simulink model "ssc_hydromech_power_split_cvt_engine_signal_intf"  (R2025a)
settings: Solver=ode23t  StartTime=0.0  StopTime=70  RelTol=1e-3  AbsTol=1e-3
StartFcn:
  | tic
StopFcn:
  | Elapsed_Sim_Time = toc;
  | disp(['Elapsed Sim Time = ' num2str(Elapsed_Sim_Time)]);
undefined symbols (not defined in the file): DiscIntNeverNeededParam, HMPST, K, Lambda, tau, x0
libraries: fl_lib x30, nesl_utility x16, sm_wheel_loader_lib x9, simulink x7, simulink_extras x6, sdl_lib x3
(part 2 of 4)

== system ssc_hydromech_power_split_cvt_engine_signal_intf/CVT/Other/CVT Ratio Ctrl ==
  Ratio (-) : Inport
  CmdVehSpdDir : Inport  Port=2
  HRBCtrl (-) : Inport  Port=3
  MBCtrl (-) : Inport  Port=4
  Bus Creator : BusCreator  Inputs=12
  Clutch Truth Table : Stateflow chart  TreatAsAtomicUnit=on
  Filter : StateSpace  A=-200  C=200  D=0  InitialCondition=HMPST.Ctrl.Swash.XY_A(1,1)/200
  Range Calculation : Subsystem  mask{XY_I=HMPST.Ctrl.Swash.XY_I}
      mask prompts: XY_I "Range Separation Points"
  Saturation : Saturate  UpperLimit=HMPST.DesignReq.MaxCVTOutputSpeed/HMPST.Eng.wTarget  LowerLimit=0  ZeroCross=off
  Swash Ctrl : Lookup_n-D  NumberOfTableDimensions=1  BreakpointsForDimension1=HMPST.Ctrl.Swash.XY_A(:,2)  BeginIndexSearchUsingPreviousIndexResult=on  Table=HMPST.Ctrl.Swash.XY_A(:,1)  InternalRulePriority=Speed  RndMeth=Simplest
  Transfer Fcn : TransferFcn  Denominator=[0.1 1]
  CVT Ctrl : Outport
  wires:
  Ratio (-)/1 -> [ratio], Transfer Fcn/1
  Clutch Truth Table/1(K1Actv) -> Bus Creator/1  "K1"
  Clutch Truth Table/2(K2Actv) -> Bus Creator/2  "K2"
  Clutch Truth Table/3(K3Actv) -> Bus Creator/3  "K3"
  Clutch Truth Table/4(K4Actv) -> Bus Creator/4  "K4"
  Clutch Truth Table/5(KbActv) -> Bus Creator/5  "Kb"
  Clutch Truth Table/6(KvActv) -> Bus Creator/6  "Kv"
  Clutch Truth Table/7(KrActv) -> Bus Creator/7  "Kr"
  Bus Creator/1 -> CVT Ctrl/1  "Ctrl"
  Range Calculation/1(Range (-)) -> Clutch Truth Table/1(Range)
  Saturation/1 -> Range Calculation/1(Ratio (-)), Swash Ctrl/1
  Transfer Fcn/1 -> Saturation/1
  Filter/1 -> Bus Creator/12  "SwashCtrl"
  Swash Ctrl/1 -> Filter/1  "SwashCtrl"
  HRBCtrl (-)/1 -> Bus Creator/8  "HRBCtrl"
  MBCtrl (-)/1 -> Bus Creator/9  "MBCtrl"
  CmdVehSpdDir/1 -> Bus Creator/11, Clutch Truth Table/2(CmdVehSpdDir)  "CmdVehSpdDir"
  [ratio] -> Bus Creator/10  "ratio"

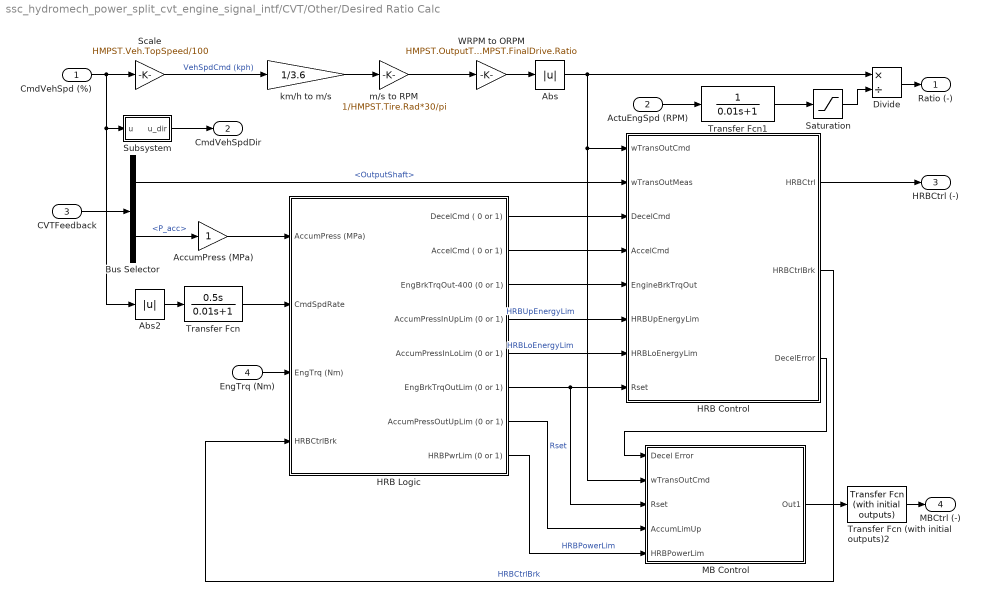
== system ssc_hydromech_power_split_cvt_engine_signal_intf/CVT/Other/Desired Ratio Calc ==
  CmdVehSpd (%) : Inport  SampleTime=HMPST.Simu.TimeStep
  ActuEngSpd (RPM) : Inport  Port=2
  CVTFeedback : Inport  Port=3
  EngTrq (Nm) : Inport  Port=4
  Abs : Abs  ZeroCross=off  SaturateOnIntegerOverflow=off
  Abs2 : Abs  ZeroCross=off  SaturateOnIntegerOverflow=off
  AccumPress (MPa) : Gain
  Bus Selector : BusSelector  OutputSignals=OutputShaft,P_acc
  Divide : Product  Inputs=*/
  HRB Control : Subsystem
  HRB Logic : Subsystem
  MB Control : Subsystem
  Saturation : Saturate  UpperLimit=2500  LowerLimit=0.5
  Scale : Gain  Gain=HMPST.Veh.TopSpeed/100
  Subsystem : Subsystem
  Transfer Fcn : TransferFcn  Numerator=[0.5 0]  Denominator=[0.01 1]
  Transfer Fcn (with initial outputs)2 : simulink_extras/Additional Linear/Transfer Fcn (with initial outputs)  N=1  D=[0.05 1]  Y0=1  U0=1
  Transfer Fcn1 : TransferFcn  Denominator=[0.01 1]
  WRPM to ORPM : Gain  Gain=HMPST.OutputTransferGearPair.Ratio*HMPST.Differential.Ratio*HMPST.FinalDrive.Ratio
  km/h to m/s : Gain  Gain=1/3.6
  m/s to RPM : Gain  Gain=1/HMPST.Tire.Rad*30/pi
  Ratio (-) : Outport
  CmdVehSpdDir : Outport  Port=2
  HRBCtrl (-) : Outport  Port=3
  MBCtrl (-) : Outport  Port=4
  wires:
  MB Control/1(Out1) -> Transfer Fcn (with initial outputs)2/1
  HRB Logic/8(HRBPwrLim (0 or 1)) -> MB Control/5(HRBPowerLim)  "HRBPowerLim"
  HRB Logic/7(AccumPressOutUpLim (0 or 1)) -> MB Control/4(AccumLimUp)
  HRB Control/3(DecelError) -> MB Control/1(Decel Error)
  HRB Control/1(HRBCtrl) -> HRBCtrl (-)/1
  HRB Logic/3(EngBrkTrqOut-400 (0 or 1)) -> HRB Control/5(EngineBrkTrqOut)
  HRB Logic/2(AccelCmd ( 0 or 1)) -> HRB Control/4(AccelCmd)
  HRB Logic/5(AccumPressInLoLim (0 or 1)) -> HRB Control/7(HRBLoEnergyLim)  "HRBLoEnergyLim"
  HRB Logic/4(AccumPressInUpLim (0 or 1)) -> HRB Control/6(HRBUpEnergyLim)  "HRBUpEnergyLim"
  HRB Logic/1(DecelCmd ( 0 or 1)) -> HRB Control/3(DecelCmd)
  Divide/1 -> Ratio (-)/1
  ActuEngSpd (RPM)/1 -> Transfer Fcn1/1
  m/s to RPM/1 -> WRPM to ORPM/1
  km/h to m/s/1 -> m/s to RPM/1
  WRPM to ORPM/1 -> Abs/1
  CmdVehSpd (%)/1 -> Abs2/1, Subsystem/1(u), Scale/1
  Saturation/1 -> Divide/2
  Transfer Fcn1/1 -> Saturation/1
  Bus Selector/1 -> HRB Control/2(wTransOutMeas)  "<OutputShaft>"
  Transfer Fcn/1 -> HRB Logic/2(CmdSpdRate)
  CVTFeedback/1 -> Bus Selector/1
  HRB Logic/6(EngBrkTrqOutLim (0 or 1)) -> MB Control/3(Rset), HRB Control/8(Rset)  "Rset"
  Bus Selector/2 -> AccumPress (MPa)/1  "<P_acc>"
  EngTrq (Nm)/1 -> HRB Logic/3(EngTrq (Nm))
  AccumPress (MPa)/1 -> HRB Logic/1(AccumPress (MPa))
  Subsystem/1(u_dir) -> CmdVehSpdDir/1
  Scale/1 -> km/h to m/s/1  "VehSpdCmd (kph)"
  Abs2/1 -> Transfer Fcn/1
  Abs/1 -> Divide/1, MB Control/2(wTransOutCmd), HRB Control/1(wTransOutCmd)
  Transfer Fcn (with initial outputs)2/1 -> MBCtrl (-)/1
  HRB Control/2(HRBCtrlBrk) -> HRB Logic/4(HRBCtrlBrk)  "HRBCtrlBrk"

== system ssc_hydromech_power_split_cvt_engine_signal_intf/CVT/Other/Port 1 Interface Engine ==
  speed : Inport
  Ideal Rotational Motion Sensor1 : fl_lib/Mechanical/Mechanical Sensors/Ideal Rotational Motion Sensor  reference=foundation.enum.MeasurementReference.difference  acceleration_port=false  velocity_port=true  position_port=true  wrap_angle=simscape.enum.onoff.off  offset=0 rad
  Interface : Subsystem  Variant=on  VariantControlMode=label  VariantControl=Variant1  LabelModeActiveChoice=Continuous
      settings: PortSchema="{\"entries\":[{\"content\":{\"sides\":[{\"content\":{\"connectorIds\":[\"In1\",\"Out2\"]},\"type\":\"ConnectorPlacement.EquallySpacedRectSide\",\"uuid\":\"aa56821c-7799-44e3-b228-553c5b43a68d\"},{\"content\":{\"connectorIds\":[\"In2\",\"Out1\"],\"side\":\"RIGHT\"},\"type\":\"ConnectorPlacement.EquallySpacedRectSide\",\"uuid\":\"8658dee5-55e2-4f33-bdec-e6600ce27fc1\"},{\"content\":{\"connectorIds\":[],\"side\":\"TOP\"},\"type\":\"ConnectorPlacement.EquallySpacedRectSide\",\"uuid\":\"2effe9c6-8e61-4f0c-a39b-329d9ffc707d\"}]},\"type\":\"ConnectorPlacement.EquallySpacedConnector\",\"uuid\":\"c8fc8444-dfc7-49a5-9550-b957635f7d8f\"}],\"packageUris\":[\"http://schema.mathworks.com/mf0/Connector/R2020b\"],\"version\":\"1.0\"}"
  Mechanical Rotational Reference2 : fl_lib/Mechanical/Rotational Elements/Mechanical Rotational Reference
  Mechanical Rotational Reference3 : fl_lib/Mechanical/Rotational Elements/Mechanical Rotational Reference
  T1 : nesl_utility/Simulink-PS Converter  PhysicalDomain=network_engine_domain  SubClassName=ps_input  LeftPortType=input  RightPortType=output  PseudoPeriodic=off  Frequencies=[]  NoiseDistribution=none  NoiseParameters=[]  Unit=N*m  AffineConversion=off  FilteringAndDerivatives=zero  SimscapeFilterOrder=1  InputFilterTimeConstant=0.001  UdotUserProvided=1
  Tau1 : fl_lib/Mechanical/Mechanical Sources/Ideal Torque Source
  w1 : nesl_utility/PS-Simulink Converter  PhysicalDomain=network_engine_domain  SubClassName=ps_output  LeftPortType=input  RightPortType=output  PseudoPeriodic=off  Frequencies=[]  VectorFormat=1-D array  Unit=rad/s  AffineConversion=off
  1 : PMIOPort  Side=Left
  torque : Outport
  wires:
  speed/1 -> Interface/2(across2)
  Interface/2(through1) -> T1/1
  w1/1 -> Interface/1(across1)
  Interface/1(through2) -> torque/1
  connections:
  1/RConn1 -- Ideal Rotational Motion Sensor1/LConn1 -- Tau1/RConn2
  Mechanical Rotational Reference2/LConn1 -- Ideal Rotational Motion Sensor1/RConn1
  Ideal Rotational Motion Sensor1/RConn2 -- w1/LConn1
  Mechanical Rotational Reference3/LConn1 -- Tau1/LConn1
  T1/RConn1 -- Tau1/RConn1

== system ssc_hydromech_power_split_cvt_engine_signal_intf/CVT/Other/Port 1 Interface Vehicle ==
  speed : Inport
  Ideal Rotational Motion Sensor1 : fl_lib/Mechanical/Mechanical Sensors/Ideal Rotational Motion Sensor  reference=foundation.enum.MeasurementReference.difference  acceleration_port=false  velocity_port=true  position_port=true  wrap_angle=simscape.enum.onoff.off  offset=0 rad
  Interface : Subsystem  Variant=on  VariantControlMode=label  VariantControl=Variant1  LabelModeActiveChoice=Continuous
      settings: PortSchema="{\"entries\":[{\"content\":{\"sides\":[{\"content\":{\"connectorIds\":[\"In1\",\"Out2\"]},\"type\":\"ConnectorPlacement.EquallySpacedRectSide\",\"uuid\":\"aa56821c-7799-44e3-b228-553c5b43a68d\"},{\"content\":{\"connectorIds\":[\"In2\",\"Out1\"],\"side\":\"RIGHT\"},\"type\":\"ConnectorPlacement.EquallySpacedRectSide\",\"uuid\":\"8658dee5-55e2-4f33-bdec-e6600ce27fc1\"},{\"content\":{\"connectorIds\":[],\"side\":\"TOP\"},\"type\":\"ConnectorPlacement.EquallySpacedRectSide\",\"uuid\":\"2effe9c6-8e61-4f0c-a39b-329d9ffc707d\"}]},\"type\":\"ConnectorPlacement.EquallySpacedConnector\",\"uuid\":\"c8fc8444-dfc7-49a5-9550-b957635f7d8f\"}],\"packageUris\":[\"http://schema.mathworks.com/mf0/Connector/R2020b\"],\"version\":\"1.0\"}"
  Mechanical Rotational Reference2 : fl_lib/Mechanical/Rotational Elements/Mechanical Rotational Reference
  Mechanical Rotational Reference3 : fl_lib/Mechanical/Rotational Elements/Mechanical Rotational Reference
  T1 : nesl_utility/Simulink-PS Converter  PhysicalDomain=network_engine_domain  SubClassName=ps_input  LeftPortType=input  RightPortType=output  PseudoPeriodic=off  Frequencies=[]  NoiseDistribution=none  NoiseParameters=[]  Unit=N*m  AffineConversion=off  FilteringAndDerivatives=zero  SimscapeFilterOrder=1  InputFilterTimeConstant=0.001  UdotUserProvided=1
  Tau1 : fl_lib/Mechanical/Mechanical Sources/Ideal Torque Source
  w1 : nesl_utility/PS-Simulink Converter  PhysicalDomain=network_engine_domain  SubClassName=ps_output  LeftPortType=input  RightPortType=output  PseudoPeriodic=off  Frequencies=[]  VectorFormat=1-D array  Unit=rad/s  AffineConversion=off
  1 : PMIOPort  Side=Left
  torque : Outport
  wires:
  speed/1 -> Interface/2(across2)
  Interface/2(through1) -> T1/1
  w1/1 -> Interface/1(across1)
  Interface/1(through2) -> torque/1
  connections:
  1/RConn1 -- Ideal Rotational Motion Sensor1/LConn1 -- Tau1/RConn2
  Mechanical Rotational Reference2/LConn1 -- Ideal Rotational Motion Sensor1/RConn1
  Ideal Rotational Motion Sensor1/RConn2 -- w1/LConn1
  Mechanical Rotational Reference3/LConn1 -- Tau1/LConn1
  T1/RConn1 -- Tau1/RConn1

== system ssc_hydromech_power_split_cvt_engine_signal_intf/CVT/Other/Power Sensor1 Engine Out ==
  Mechanical Rotational Reference : fl_lib/Mechanical/Rotational Elements/Mechanical Rotational Reference
  PS Terminator : fl_lib/Physical Signals/Sinks/PS Terminator
  Power Sensor : sdl_lib/Sensors/Rotational Power Sensor  measurement_type=sdl.enum.rotationalPowerSensorType.instantaneous  averaging_period=1 s  max_frequency=1000 Hz  max_speed=1000 rpm
      settings: InternalSimscapePortConfiguration="{\"Bottom\":[],\"Left\":[{\"id\":\"S\",\"label\":\"S\",\"type\":\"foundation.mechanical.rotational.rotational\"},{\"id\":\"R\",\"label\":\"R\",\"type\":\"foundation.mechanical.rotational.rotational\"},{\"id\":\"C\",\"label\":\"C\",\"type\":\"foundation.mechanical.rotational.rotational\"}],\"Right\":[{\"id\":\"P\",\"label\":\"P\",\"type\":\"output\"}],\"Top\":[]}"
  S : PMIOPort  Side=Left
  R : PMIOPort  Port=2  Side=Right
  connections:
  Power Sensor/LConn1 -- S/RConn1
  Power Sensor/LConn2 -- R/RConn1
  Power Sensor/LConn3 -- Mechanical Rotational Reference/LConn1
  Power Sensor/RConn1 -- PS Terminator/LConn1

== system ssc_hydromech_power_split_cvt_engine_signal_intf/CVT/Other/Scopes ==
  CVTCtrl : Inport
  mCVT : Inport  Port=2
  Bus Selector1 : BusSelector  OutputSignals=wIn,OutputShaft
  Bus Selector2 : BusSelector  OutputSignals=K1,K2,K3,K4,Kb,Kv,Kr
  Bus Selector3 : BusSelector  OutputSignals=SwashCtrl,HRBCtrl,MBCtrl
  CVT Ctrl : Scope
      settings: ActiveDisplayYMinimum=-0.96987  ActiveDisplayYMaximum=1.21887  DataLoggingVariableName=ScopeData2
  Scope : Scope  NumInputPorts=2
      settings: ActiveDisplayYMinimum=-1460.02488  ActiveDisplayYMaximum=1460.04785  DataLoggingVariableName=ScopeData4
  Scope1 : Scope  NumInputPorts=7
      settings: ActiveDisplayYMinimum=-0.125  ActiveDisplayYMaximum=1.125  DataLoggingVariableName=ScopeData3
  Scope2 : Scope  NumInputPorts=3
      settings: ActiveDisplayYMinimum=-0.96987  ActiveDisplayYMaximum=1.21887  DataLoggingVariableName=ScopeData4
  wires:
  Bus Selector2/7 -> Scope1/7  "<Kr>"
  Bus Selector2/5 -> Scope1/5  "<Kb>"
  Bus Selector2/4 -> Scope1/4  "<K4>"
  Bus Selector3/3 -> Scope2/3  "<MBCtrl>"
  Bus Selector3/1 -> Scope2/1  "<SwashCtrl>"
  Bus Selector2/2 -> Scope1/2  "<K2>"
  Bus Selector2/6 -> Scope1/6  "<Kv>"
  Bus Selector2/3 -> Scope1/3  "<K3>"
  Bus Selector3/2 -> Scope2/2  "<HRBCtrl>"
  CVTCtrl/1 -> Bus Selector2/1, CVT Ctrl/1, Bus Selector3/1
  Bus Selector2/1 -> Scope1/1  "<K1>"
  mCVT/1 -> Bus Selector1/1
  Bus Selector1/2 -> Scope/2  "<OutputShaft>"
  Bus Selector1/1 -> Scope/1  "<wIn>"

== system ssc_hydromech_power_split_cvt_engine_signal_intf/CVT/Other/Transmission ==
  Ctrl : Inport
  Abstract : sm_wheel_loader_lib/CVT Abstract  VariantControl=Abstract  dShaftE=HMPST.AbstractCVT.dInput  dShaftD=HMPST.AbstractCVT.dOutput  k=HMPST.AbstractCVT.kCompliance  d=HMPST.AbstractCVT.dCompliance
  Hydrostatic : sm_wheel_loader_lib/Hydrostatic  SystemSampleTime=-1  VariantControl=Hydrostatic  VariantActivationTime=update diagram  EmptyChoice=off  PassThrough=off  PassThroughVariantControl=(default)  EmptyChoiceVariantControl=(default)  AllowFlexibleInterface=on  Latency=0  AutoFrameSizeCalculation=off
  Power Split Hydromech : sm_wheel_loader_lib/CVT Power Split Hydromechanical  SystemSampleTime=-1  VariantControl=Power_Split_HM  VariantActivationTime=update diagram  EmptyChoice=off  PassThrough=off  PassThroughVariantControl=(default)  EmptyChoiceVariantControl=(default)  AllowFlexibleInterface=on  Latency=0  AutoFrameSizeCalculation=off
      settings: LibrarySourceBlock=sm_wheel_loader_lib/CVT Powersplit Hydromechanical
  E : PMIOPort  Side=Left
  D : PMIOPort  Port=2  Side=Right
  m : Outport

== system ssc_hydromech_power_split_cvt_engine_signal_intf/CVT/Simscape/CVT Ratio Ctrl ==
  Ratio (-) : Inport
  CmdVehSpdDir : Inport  Port=2
  HRBCtrl (-) : Inport  Port=3
  MBCtrl (-) : Inport  Port=4
  Bus Creator : BusCreator  Inputs=12
  Clutch Truth Table : Stateflow chart  TreatAsAtomicUnit=on
  Filter : StateSpace  A=-200  C=200  D=0  InitialCondition=HMPST.Ctrl.Swash.XY_A(1,1)/200
  Range Calculation : Subsystem  mask{XY_I=HMPST.Ctrl.Swash.XY_I}
      mask prompts: XY_I "Range Separation Points"
  Saturation : Saturate  UpperLimit=HMPST.DesignReq.MaxCVTOutputSpeed/HMPST.Eng.wTarget  LowerLimit=0  ZeroCross=off
  Swash Ctrl : Lookup_n-D  NumberOfTableDimensions=1  BreakpointsForDimension1=HMPST.Ctrl.Swash.XY_A(:,2)  BeginIndexSearchUsingPreviousIndexResult=on  Table=HMPST.Ctrl.Swash.XY_A(:,1)  InternalRulePriority=Speed  RndMeth=Simplest
  Transfer Fcn : TransferFcn  Denominator=[0.1 1]
  CVT Ctrl : Outport
  wires:
  [ratio] -> Bus Creator/10  "ratio"
  CmdVehSpdDir/1 -> Clutch Truth Table/2(CmdVehSpdDir), Bus Creator/11  "CmdVehSpdDir"
  MBCtrl (-)/1 -> Bus Creator/9  "MBCtrl"
  HRBCtrl (-)/1 -> Bus Creator/8  "HRBCtrl"
  Swash Ctrl/1 -> Filter/1  "SwashCtrl"
  Filter/1 -> Bus Creator/12  "SwashCtrl"
  Transfer Fcn/1 -> Saturation/1
  Saturation/1 -> Swash Ctrl/1, Range Calculation/1(Ratio (-))
  Range Calculation/1(Range (-)) -> Clutch Truth Table/1(Range)
  Bus Creator/1 -> CVT Ctrl/1  "Ctrl"
  Clutch Truth Table/7(KrActv) -> Bus Creator/7  "Kr"
  Clutch Truth Table/6(KvActv) -> Bus Creator/6  "Kv"
  Clutch Truth Table/5(KbActv) -> Bus Creator/5  "Kb"
  Clutch Truth Table/4(K4Actv) -> Bus Creator/4  "K4"
  Clutch Truth Table/3(K3Actv) -> Bus Creator/3  "K3"
  Clutch Truth Table/2(K2Actv) -> Bus Creator/2  "K2"
  Clutch Truth Table/1(K1Actv) -> Bus Creator/1  "K1"
  Ratio (-)/1 -> Transfer Fcn/1, [ratio]

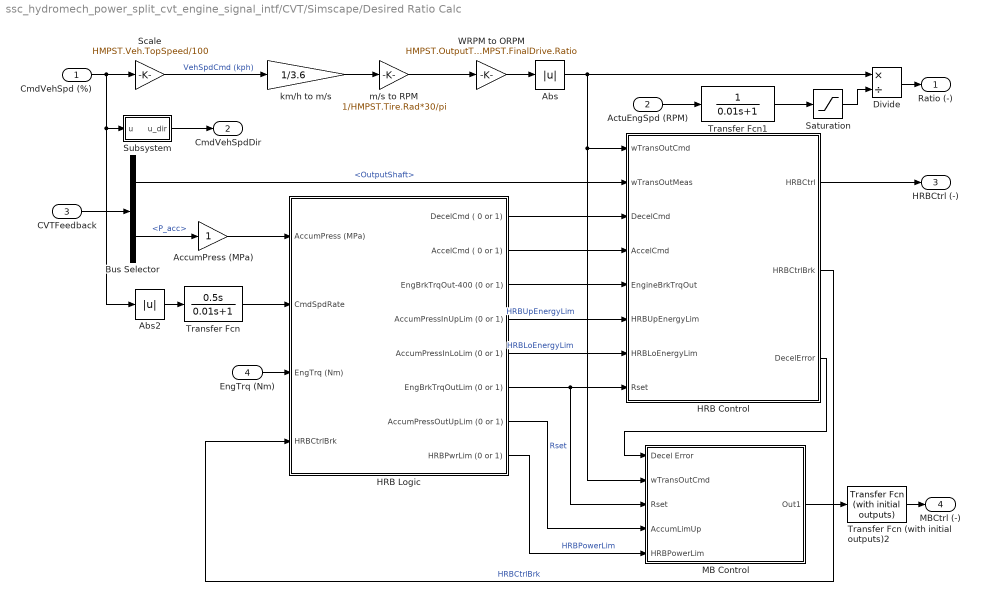
== system ssc_hydromech_power_split_cvt_engine_signal_intf/CVT/Simscape/Desired Ratio Calc ==
  CmdVehSpd (%) : Inport  SampleTime=HMPST.Simu.TimeStep
  ActuEngSpd (RPM) : Inport  Port=2
  CVTFeedback : Inport  Port=3
  EngTrq (Nm) : Inport  Port=4
  Abs : Abs  ZeroCross=off  SaturateOnIntegerOverflow=off
  Abs2 : Abs  ZeroCross=off  SaturateOnIntegerOverflow=off
  AccumPress (MPa) : Gain
  Bus Selector : BusSelector  OutputSignals=OutputShaft,P_acc
  Divide : Product  Inputs=*/
  HRB Control : Subsystem
  HRB Logic : Subsystem
  MB Control : Subsystem
  Saturation : Saturate  UpperLimit=2500  LowerLimit=0.5
  Scale : Gain  Gain=HMPST.Veh.TopSpeed/100
  Subsystem : Subsystem
  Transfer Fcn : TransferFcn  Numerator=[0.5 0]  Denominator=[0.01 1]
  Transfer Fcn (with initial outputs)2 : simulink_extras/Additional Linear/Transfer Fcn (with initial outputs)  N=1  D=[0.05 1]  Y0=1  U0=1
  Transfer Fcn1 : TransferFcn  Denominator=[0.01 1]
  WRPM to ORPM : Gain  Gain=HMPST.OutputTransferGearPair.Ratio*HMPST.Differential.Ratio*HMPST.FinalDrive.Ratio
  km/h to m/s : Gain  Gain=1/3.6
  m/s to RPM : Gain  Gain=1/HMPST.Tire.Rad*30/pi
  Ratio (-) : Outport
  CmdVehSpdDir : Outport  Port=2
  HRBCtrl (-) : Outport  Port=3
  MBCtrl (-) : Outport  Port=4
  wires:
  HRB Control/2(HRBCtrlBrk) -> HRB Logic/4(HRBCtrlBrk)  "HRBCtrlBrk"
  Transfer Fcn (with initial outputs)2/1 -> MBCtrl (-)/1
  Abs/1 -> HRB Control/1(wTransOutCmd), MB Control/2(wTransOutCmd), Divide/1
  Abs2/1 -> Transfer Fcn/1
  Scale/1 -> km/h to m/s/1  "VehSpdCmd (kph)"
  Subsystem/1(u_dir) -> CmdVehSpdDir/1
  AccumPress (MPa)/1 -> HRB Logic/1(AccumPress (MPa))
  EngTrq (Nm)/1 -> HRB Logic/3(EngTrq (Nm))
  Bus Selector/2 -> AccumPress (MPa)/1  "<P_acc>"
  HRB Logic/6(EngBrkTrqOutLim (0 or 1)) -> HRB Control/8(Rset), MB Control/3(Rset)  "Rset"
  CVTFeedback/1 -> Bus Selector/1
  Transfer Fcn/1 -> HRB Logic/2(CmdSpdRate)
  Bus Selector/1 -> HRB Control/2(wTransOutMeas)  "<OutputShaft>"
  Transfer Fcn1/1 -> Saturation/1
  Saturation/1 -> Divide/2
  CmdVehSpd (%)/1 -> Scale/1, Subsystem/1(u), Abs2/1
  WRPM to ORPM/1 -> Abs/1
  km/h to m/s/1 -> m/s to RPM/1
  m/s to RPM/1 -> WRPM to ORPM/1
  ActuEngSpd (RPM)/1 -> Transfer Fcn1/1
  Divide/1 -> Ratio (-)/1
  HRB Logic/1(DecelCmd ( 0 or 1)) -> HRB Control/3(DecelCmd)
  HRB Logic/4(AccumPressInUpLim (0 or 1)) -> HRB Control/6(HRBUpEnergyLim)  "HRBUpEnergyLim"
  HRB Logic/5(AccumPressInLoLim (0 or 1)) -> HRB Control/7(HRBLoEnergyLim)  "HRBLoEnergyLim"
  HRB Logic/2(AccelCmd ( 0 or 1)) -> HRB Control/4(AccelCmd)
  HRB Logic/3(EngBrkTrqOut-400 (0 or 1)) -> HRB Control/5(EngineBrkTrqOut)
  HRB Control/1(HRBCtrl) -> HRBCtrl (-)/1
  HRB Control/3(DecelError) -> MB Control/1(Decel Error)
  HRB Logic/7(AccumPressOutUpLim (0 or 1)) -> MB Control/4(AccumLimUp)
  HRB Logic/8(HRBPwrLim (0 or 1)) -> MB Control/5(HRBPowerLim)  "HRBPowerLim"
  MB Control/1(Out1) -> Transfer Fcn (with initial outputs)2/1

== system ssc_hydromech_power_split_cvt_engine_signal_intf/CVT/Simscape/Port 1 Interface Engine ==
  speed : Inport
  Ideal Rotational Motion Sensor1 : fl_lib/Mechanical/Mechanical Sensors/Ideal Rotational Motion Sensor  reference=foundation.enum.MeasurementReference.difference  acceleration_port=false  velocity_port=true  position_port=true  wrap_angle=simscape.enum.onoff.off  offset=0 rad
  Interface : Subsystem  Variant=on  VariantControlMode=label  VariantControl=Variant1  LabelModeActiveChoice=Continuous
      settings: PortSchema="{\"entries\":[{\"content\":{\"sides\":[{\"content\":{\"connectorIds\":[\"In1\",\"Out2\"]},\"type\":\"ConnectorPlacement.EquallySpacedRectSide\",\"uuid\":\"aa56821c-7799-44e3-b228-553c5b43a68d\"},{\"content\":{\"connectorIds\":[\"In2\",\"Out1\"],\"side\":\"RIGHT\"},\"type\":\"ConnectorPlacement.EquallySpacedRectSide\",\"uuid\":\"8658dee5-55e2-4f33-bdec-e6600ce27fc1\"},{\"content\":{\"connectorIds\":[],\"side\":\"TOP\"},\"type\":\"ConnectorPlacement.EquallySpacedRectSide\",\"uuid\":\"2effe9c6-8e61-4f0c-a39b-329d9ffc707d\"}]},\"type\":\"ConnectorPlacement.EquallySpacedConnector\",\"uuid\":\"c8fc8444-dfc7-49a5-9550-b957635f7d8f\"}],\"packageUris\":[\"http://schema.mathworks.com/mf0/Connector/R2020b\"],\"version\":\"1.0\"}"
  Mechanical Rotational Reference2 : fl_lib/Mechanical/Rotational Elements/Mechanical Rotational Reference
  Mechanical Rotational Reference3 : fl_lib/Mechanical/Rotational Elements/Mechanical Rotational Reference
  T1 : nesl_utility/Simulink-PS Converter  PhysicalDomain=network_engine_domain  SubClassName=ps_input  LeftPortType=input  RightPortType=output  PseudoPeriodic=off  Frequencies=[]  NoiseDistribution=none  NoiseParameters=[]  Unit=N*m  AffineConversion=off  FilteringAndDerivatives=zero  SimscapeFilterOrder=1  InputFilterTimeConstant=0.001  UdotUserProvided=1
  Tau1 : fl_lib/Mechanical/Mechanical Sources/Ideal Torque Source
  w1 : nesl_utility/PS-Simulink Converter  PhysicalDomain=network_engine_domain  SubClassName=ps_output  LeftPortType=input  RightPortType=output  PseudoPeriodic=off  Frequencies=[]  VectorFormat=1-D array  Unit=rad/s  AffineConversion=off
  1 : PMIOPort  Side=Left
  torque : Outport
  wires:
  Interface/1(through2) -> torque/1
  w1/1 -> Interface/1(across1)
  Interface/2(through1) -> T1/1
  speed/1 -> Interface/2(across2)
  connections:
  T1/RConn1 -- Tau1/RConn1
  Mechanical Rotational Reference3/LConn1 -- Tau1/LConn1
  Ideal Rotational Motion Sensor1/RConn2 -- w1/LConn1
  Mechanical Rotational Reference2/LConn1 -- Ideal Rotational Motion Sensor1/RConn1
  Tau1/RConn2 -- Ideal Rotational Motion Sensor1/LConn1 -- 1/RConn1

== system ssc_hydromech_power_split_cvt_engine_signal_intf/CVT/Simscape/Port 1 Interface Vehicle ==
  speed : Inport
  Ideal Rotational Motion Sensor1 : fl_lib/Mechanical/Mechanical Sensors/Ideal Rotational Motion Sensor  reference=foundation.enum.MeasurementReference.difference  acceleration_port=false  velocity_port=true  position_port=true  wrap_angle=simscape.enum.onoff.off  offset=0 rad
  Interface : Subsystem  Variant=on  VariantControlMode=label  VariantControl=Variant1  LabelModeActiveChoice=Continuous
      settings: PortSchema="{\"entries\":[{\"content\":{\"sides\":[{\"content\":{\"connectorIds\":[\"In1\",\"Out2\"]},\"type\":\"ConnectorPlacement.EquallySpacedRectSide\",\"uuid\":\"aa56821c-7799-44e3-b228-553c5b43a68d\"},{\"content\":{\"connectorIds\":[\"In2\",\"Out1\"],\"side\":\"RIGHT\"},\"type\":\"ConnectorPlacement.EquallySpacedRectSide\",\"uuid\":\"8658dee5-55e2-4f33-bdec-e6600ce27fc1\"},{\"content\":{\"connectorIds\":[],\"side\":\"TOP\"},\"type\":\"ConnectorPlacement.EquallySpacedRectSide\",\"uuid\":\"2effe9c6-8e61-4f0c-a39b-329d9ffc707d\"}]},\"type\":\"ConnectorPlacement.EquallySpacedConnector\",\"uuid\":\"c8fc8444-dfc7-49a5-9550-b957635f7d8f\"}],\"packageUris\":[\"http://schema.mathworks.com/mf0/Connector/R2020b\"],\"version\":\"1.0\"}"
  Mechanical Rotational Reference2 : fl_lib/Mechanical/Rotational Elements/Mechanical Rotational Reference
  Mechanical Rotational Reference3 : fl_lib/Mechanical/Rotational Elements/Mechanical Rotational Reference
  T1 : nesl_utility/Simulink-PS Converter  PhysicalDomain=network_engine_domain  SubClassName=ps_input  LeftPortType=input  RightPortType=output  PseudoPeriodic=off  Frequencies=[]  NoiseDistribution=none  NoiseParameters=[]  Unit=N*m  AffineConversion=off  FilteringAndDerivatives=zero  SimscapeFilterOrder=1  InputFilterTimeConstant=0.001  UdotUserProvided=1
  Tau1 : fl_lib/Mechanical/Mechanical Sources/Ideal Torque Source
  w1 : nesl_utility/PS-Simulink Converter  PhysicalDomain=network_engine_domain  SubClassName=ps_output  LeftPortType=input  RightPortType=output  PseudoPeriodic=off  Frequencies=[]  VectorFormat=1-D array  Unit=rad/s  AffineConversion=off
  1 : PMIOPort  Side=Left
  torque : Outport
  wires:
  Interface/1(through2) -> torque/1
  w1/1 -> Interface/1(across1)
  Interface/2(through1) -> T1/1
  speed/1 -> Interface/2(across2)
  connections:
  T1/RConn1 -- Tau1/RConn1
  Mechanical Rotational Reference3/LConn1 -- Tau1/LConn1
  Ideal Rotational Motion Sensor1/RConn2 -- w1/LConn1
  Mechanical Rotational Reference2/LConn1 -- Ideal Rotational Motion Sensor1/RConn1
  Tau1/RConn2 -- Ideal Rotational Motion Sensor1/LConn1 -- 1/RConn1

== system ssc_hydromech_power_split_cvt_engine_signal_intf/CVT/Simscape/Power Sensor1 Engine Out ==
  Mechanical Rotational Reference : fl_lib/Mechanical/Rotational Elements/Mechanical Rotational Reference
  PS Terminator : fl_lib/Physical Signals/Sinks/PS Terminator
  Power Sensor : sdl_lib/Sensors/Rotational Power Sensor  measurement_type=sdl.enum.rotationalPowerSensorType.instantaneous  averaging_period=1 s  max_frequency=1000 Hz  max_speed=1000 rpm
      settings: InternalSimscapePortConfiguration="{\"Bottom\":[],\"Left\":[{\"id\":\"S\",\"label\":\"S\",\"type\":\"foundation.mechanical.rotational.rotational\"},{\"id\":\"R\",\"label\":\"R\",\"type\":\"foundation.mechanical.rotational.rotational\"},{\"id\":\"C\",\"label\":\"C\",\"type\":\"foundation.mechanical.rotational.rotational\"}],\"Right\":[{\"id\":\"P\",\"label\":\"P\",\"type\":\"output\"}],\"Top\":[]}"
  S : PMIOPort  Side=Left
  R : PMIOPort  Port=2  Side=Right
  connections:
  Power Sensor/RConn1 -- PS Terminator/LConn1
  Power Sensor/LConn3 -- Mechanical Rotational Reference/LConn1
  Power Sensor/LConn2 -- R/RConn1
  Power Sensor/LConn1 -- S/RConn1

== system ssc_hydromech_power_split_cvt_engine_signal_intf/CVT/Simscape/Power Sensor2 CVT Out ==
  Mechanical Rotational Reference : fl_lib/Mechanical/Rotational Elements/Mechanical Rotational Reference
  PS Terminator : fl_lib/Physical Signals/Sinks/PS Terminator
  Power Sensor : sdl_lib/Sensors/Rotational Power Sensor  measurement_type=sdl.enum.rotationalPowerSensorType.instantaneous  averaging_period=1 s  max_frequency=1000 Hz  max_speed=1000 rpm
      settings: InternalSimscapePortConfiguration="{\"Bottom\":[],\"Left\":[{\"id\":\"S\",\"label\":\"S\",\"type\":\"foundation.mechanical.rotational.rotational\"},{\"id\":\"R\",\"label\":\"R\",\"type\":\"foundation.mechanical.rotational.rotational\"},{\"id\":\"C\",\"label\":\"C\",\"type\":\"foundation.mechanical.rotational.rotational\"}],\"Right\":[{\"id\":\"P\",\"label\":\"P\",\"type\":\"output\"}],\"Top\":[]}"
  S : PMIOPort  Side=Left
  R : PMIOPort  Port=2  Side=Right
  connections:
  Power Sensor/LConn1 -- S/RConn1
  Power Sensor/LConn2 -- R/RConn1
  Power Sensor/LConn3 -- Mechanical Rotational Reference/LConn1
  Power Sensor/RConn1 -- PS Terminator/LConn1

== system ssc_hydromech_power_split_cvt_engine_signal_intf/CVT/Simscape/Scopes ==
  CVTCtrl : Inport
  mCVT : Inport  Port=2
  Bus Selector1 : BusSelector  OutputSignals=wIn,OutputShaft
  Bus Selector2 : BusSelector  OutputSignals=K1,K2,K3,K4,Kb,Kv,Kr
  Bus Selector3 : BusSelector  OutputSignals=SwashCtrl,HRBCtrl,MBCtrl
  CVT Ctrl : Scope
      settings: ActiveDisplayYMinimum=-0.96987  ActiveDisplayYMaximum=1.21887  DataLoggingVariableName=ScopeData2
  Scope : Scope  NumInputPorts=2
      settings: ActiveDisplayYMinimum=-1460.02488  ActiveDisplayYMaximum=1460.04785  DataLoggingVariableName=ScopeData4
  Scope1 : Scope  NumInputPorts=7
      settings: ActiveDisplayYMinimum=-0.125  ActiveDisplayYMaximum=1.125  DataLoggingVariableName=ScopeData3
  Scope2 : Scope  NumInputPorts=3
      settings: ActiveDisplayYMinimum=-0.96987  ActiveDisplayYMaximum=1.21887  DataLoggingVariableName=ScopeData4
  wires:
  Bus Selector1/1 -> Scope/1  "<wIn>"
  Bus Selector1/2 -> Scope/2  "<OutputShaft>"
  mCVT/1 -> Bus Selector1/1
  Bus Selector2/1 -> Scope1/1  "<K1>"
  CVTCtrl/1 -> Bus Selector3/1, CVT Ctrl/1, Bus Selector2/1
  Bus Selector3/2 -> Scope2/2  "<HRBCtrl>"
  Bus Selector2/3 -> Scope1/3  "<K3>"
  Bus Selector2/6 -> Scope1/6  "<Kv>"
  Bus Selector2/2 -> Scope1/2  "<K2>"
  Bus Selector3/1 -> Scope2/1  "<SwashCtrl>"
  Bus Selector3/3 -> Scope2/3  "<MBCtrl>"
  Bus Selector2/4 -> Scope1/4  "<K4>"
  Bus Selector2/5 -> Scope1/5  "<Kb>"
  Bus Selector2/7 -> Scope1/7  "<Kr>"

== system ssc_hydromech_power_split_cvt_engine_signal_intf/CVT/Simscape/Transmission ==
  Ctrl : Inport
  Abstract : sm_wheel_loader_lib/CVT Abstract  VariantControl=Abstract  dShaftE=HMPST.AbstractCVT.dInput  dShaftD=HMPST.AbstractCVT.dOutput  k=HMPST.AbstractCVT.kCompliance  d=HMPST.AbstractCVT.dCompliance
  Hydrostatic : sm_wheel_loader_lib/Hydrostatic  SystemSampleTime=-1  VariantControl=Hydrostatic  VariantActivationTime=update diagram  EmptyChoice=off  PassThrough=off  PassThroughVariantControl=(default)  EmptyChoiceVariantControl=(default)  AllowFlexibleInterface=on  Latency=0  AutoFrameSizeCalculation=off
  Power Split Hydromech : sm_wheel_loader_lib/CVT Power Split Hydromechanical  SystemSampleTime=-1  VariantControl=Power_Split_HM  VariantActivationTime=update diagram  EmptyChoice=off  PassThrough=off  PassThroughVariantControl=(default)  EmptyChoiceVariantControl=(default)  AllowFlexibleInterface=on  Latency=0  AutoFrameSizeCalculation=off
      settings: LibrarySourceBlock=sm_wheel_loader_lib/CVT Powersplit Hydromechanical
  E : PMIOPort  Side=Left
  D : PMIOPort  Port=2  Side=Right
  m : Outport

== system ssc_hydromech_power_split_cvt_engine_signal_intf/Engine/Simscape/Port 2 Interface ==
  torque : Inport
  Ideal Rotational Motion Sensor2 : fl_lib/Mechanical/Mechanical Sensors/Ideal Rotational Motion Sensor  reference=foundation.enum.MeasurementReference.difference  acceleration_port=false  velocity_port=true  position_port=true  wrap_angle=simscape.enum.onoff.off  offset=0 rad
  Mechanical Rotational Reference1 : fl_lib/Mechanical/Rotational Elements/Mechanical Rotational Reference
  Mechanical Rotational Reference4 : fl_lib/Mechanical/Rotational Elements/Mechanical Rotational Reference
  T2 : nesl_utility/Simulink-PS Converter  PhysicalDomain=network_engine_domain  SubClassName=ps_input  LeftPortType=input  RightPortType=output  PseudoPeriodic=off  Frequencies=[]  NoiseDistribution=none  NoiseParameters=[]  Unit=N*m  AffineConversion=off  FilteringAndDerivatives=zero  SimscapeFilterOrder=1  InputFilterTimeConstant=0.001  UdotUserProvided=1
  Tau2 : fl_lib/Mechanical/Mechanical Sources/Ideal Torque Source
  w2 : nesl_utility/PS-Simulink Converter  PhysicalDomain=network_engine_domain  SubClassName=ps_output  LeftPortType=input  RightPortType=output  PseudoPeriodic=off  Frequencies=[]  VectorFormat=1-D array  Unit=rpm  AffineConversion=off
  2 : PMIOPort  Side=Right
  speed : Outport
  wires:
  w2/1 -> speed/1
  torque/1 -> T2/1
  connections:
  Mechanical Rotational Reference4/LConn1 -- Tau2/LConn1
  Tau2/RConn2 -- 2/RConn1 -- Ideal Rotational Motion Sensor2/LConn1
  Ideal Rotational Motion Sensor2/RConn2 -- w2/LConn1
  Mechanical Rotational Reference1/LConn1 -- Ideal Rotational Motion Sensor2/RConn1
  T2/RConn1 -- Tau2/RConn1

== system ssc_hydromech_power_split_cvt_engine_signal_intf/Vehicle/Simscape/Port 2 Interface Vehicle ==
  torque : Inport
  Ideal Rotational Motion Sensor2 : fl_lib/Mechanical/Mechanical Sensors/Ideal Rotational Motion Sensor  reference=foundation.enum.MeasurementReference.difference  acceleration_port=false  velocity_port=true  position_port=true  wrap_angle=simscape.enum.onoff.off  offset=0 rad
  Mechanical Rotational Reference1 : fl_lib/Mechanical/Rotational Elements/Mechanical Rotational Reference
  Mechanical Rotational Reference4 : fl_lib/Mechanical/Rotational Elements/Mechanical Rotational Reference
  T2 : nesl_utility/Simulink-PS Converter  PhysicalDomain=network_engine_domain  SubClassName=ps_input  LeftPortType=input  RightPortType=output  PseudoPeriodic=off  Frequencies=[]  NoiseDistribution=none  NoiseParameters=[]  Unit=N*m  AffineConversion=off  FilteringAndDerivatives=zero  SimscapeFilterOrder=1  InputFilterTimeConstant=0.001  UdotUserProvided=1
  Tau2 : fl_lib/Mechanical/Mechanical Sources/Ideal Torque Source
  w2 : nesl_utility/PS-Simulink Converter  PhysicalDomain=network_engine_domain  SubClassName=ps_output  LeftPortType=input  RightPortType=output  PseudoPeriodic=off  Frequencies=[]  VectorFormat=1-D array  Unit=rpm  AffineConversion=off
  2 : PMIOPort  Side=Right
  speed : Outport
  wires:
  w2/1 -> speed/1
  torque/1 -> T2/1
  connections:
  Mechanical Rotational Reference4/LConn1 -- Tau2/LConn1
  Tau2/RConn2 -- 2/RConn1 -- Ideal Rotational Motion Sensor2/LConn1
  Ideal Rotational Motion Sensor2/RConn2 -- w2/LConn1
  Mechanical Rotational Reference1/LConn1 -- Ideal Rotational Motion Sensor2/RConn1
  T2/RConn1 -- Tau2/RConn1

== system ssc_hydromech_power_split_cvt_engine_signal_intf/Vehicle/Simscape/Vehicle ==
  Driveline : sm_wheel_loader_lib/Wheel Loader Vehicle/Driveline/Driveline/Driveline 1D/Driveline  SystemSampleTime=-1  VariantActivationTime=update diagram  EmptyChoice=off  PassThrough=off  PassThroughVariantControl=(default)  EmptyChoiceVariantControl=(default)  AllowFlexibleInterface=on  Latency=0  AutoFrameSizeCalculation=off
  Tires and Body : sm_wheel_loader_lib/Tires and Body 1D  SystemSampleTime=-1  VariantActivationTime=update diagram  EmptyChoice=off  PassThrough=off  PassThroughVariantControl=(default)  EmptyChoiceVariantControl=(default)  AllowFlexibleInterface=on  Latency=0  AutoFrameSizeCalculation=off
      settings: PortSchema="{\"entries\":[{\"content\":{\"sides\":[{\"content\":{\"connectorIds\":[\"LConn1\",\"LConn2\"]},\"type\":\"ConnectorPlacement.EquallySpacedRectSide\",\"uuid\":\"f6e4eca3-fb02-4523-87a7-c8328825f67f\"},{\"content\":{\"connectorIds\":[\"RConn1\",\"RConn2\"],\"side\":\"RIGHT\"},\"type\":\"ConnectorPlacement.EquallySpacedRectSide\",\"uuid\":\"a01e7d42-3992-448e-add1-f2755d8f064c\"},{\"content\":{\"connectorIds\":[\"Out1\"],\"side\":\"TOP\"},\"type\":\"ConnectorPlacement.EquallySpacedRectSide\",\"uuid\":\"cf483cf6-51ef-4c82-b2ec-fd42745a5c51\"},{\"content\":{\"side\":\"BOTTOM\"},\"type\":\"ConnectorPlacement.EquallySpacedRectSide\",\"uuid\":\"9bbb772c-3b9f-4e30-8c40-373d820ff5eb\"}]},\"type\":\"ConnectorPlacement.EquallySpacedConnector\",\"uuid\":\"52398d34-f462-4e1c-abff-1dda3b221c82\"}],\"packageUris\":[\"http://schema.mathworks.com/mf0/Connector/R2020b\"],\"version\":\"1.0\"}"
  Tr : PMIOPort  Side=Left
  v : Outport
  wires:
  Tires and Body/1 -> v/1
  connections:
  Tires and Body/LConn1 -- Driveline/LConn3
  Tires and Body/LConn2 -- Driveline/LConn1
  Driveline/RConn3 -- Tires and Body/RConn1
  Driveline/RConn1 -- Tires and Body/RConn2
  Tr/RConn1 -- Driveline/RConn2

== system ssc_hydromech_power_split_cvt_engine_signal_intf/CVT/Other/CVT Ratio Ctrl/Range Calculation ==
  Ratio (-) : Inport
  Check Range 0 or higher : Switch  Threshold=XY_I(1,2)  SaturateOnIntegerOverflow=off  InputSameDT=off
  Check Range 2 or higher : Switch  Threshold=XY_I(2,2)  SaturateOnIntegerOverflow=off  InputSameDT=off
  Check Range 3 or higher : Switch  Threshold=XY_I(3,2)  SaturateOnIntegerOverflow=off  InputSameDT=off
  Check Range 4 : Switch  Threshold=XY_I(4,2)  SaturateOnIntegerOverflow=off  InputSameDT=off
  Constant1 : Constant  Value=2  SampleTime=HMPST.Simu.TimeStep
  Constant2 : Constant  SampleTime=HMPST.Simu.TimeStep
  Constant3 : Constant  Value=-1  SampleTime=HMPST.Simu.TimeStep
  Constant4 : Constant  Value=3  SampleTime=HMPST.Simu.TimeStep
  Constant5 : Constant  Value=4  SampleTime=HMPST.Simu.TimeStep
  Range (-) : Outport
  wires:
  Check Range 2 or higher/1 -> Check Range 0 or higher/1
  Constant2/1 -> Check Range 2 or higher/3
  Constant3/1 -> Check Range 0 or higher/3
  Check Range 0 or higher/1 -> Range (-)/1  "Range"
  Check Range 3 or higher/1 -> Check Range 2 or higher/1
  Constant1/1 -> Check Range 3 or higher/3
  Check Range 4/1 -> Check Range 3 or higher/1
  Constant4/1 -> Check Range 4/3
  Constant5/1 -> Check Range 4/1
  Ratio (-)/1 -> Check Range 2 or higher/2, Check Range 3 or higher/2, Check Range 4/2, Check Range 0 or higher/2

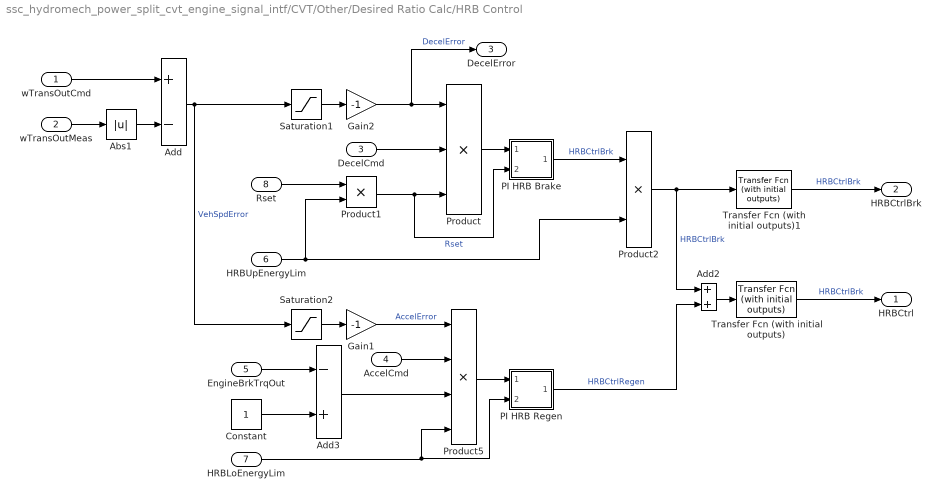
== system ssc_hydromech_power_split_cvt_engine_signal_intf/CVT/Other/Desired Ratio Calc/HRB Control ==
  wTransOutCmd : Inport
  wTransOutMeas : Inport  Port=2
  DecelCmd : Inport  Port=3
  AccelCmd : Inport  Port=4
  EngineBrkTrqOut : Inport  Port=5
  HRBUpEnergyLim : Inport  Port=6
  HRBLoEnergyLim : Inport  Port=7
  Rset : Inport  Port=8
  Abs1 : Abs  ZeroCross=off  SaturateOnIntegerOverflow=off
  Add : Sum  Inputs=+-
  Add2 : Sum
  Add3 : Sum  Inputs=-+
  Constant : Constant
  Gain1 : Gain  Gain=-1
  Gain2 : Gain  Gain=-1
  PI HRB Brake : Subsystem
  PI HRB Regen : Subsystem
  Product : Product  Inputs=3
  Product1 : Product
  Product2 : Product
  Product5 : Product  Inputs=4
  Saturation1 : Saturate  UpperLimit=0  LowerLimit=-inf  ZeroCross=off
  Saturation2 : Saturate  UpperLimit=inf  LowerLimit=0  ZeroCross=off
  Transfer Fcn (with initial outputs) : simulink_extras/Additional Linear/Transfer Fcn (with initial outputs)  N=[0.01]  D=[0.05 1]  Y0=0  U0=0
  Transfer Fcn (with initial outputs)1 : simulink_extras/Additional Linear/Transfer Fcn (with initial outputs)  N=[0.01]  D=[0.05 1]  Y0=0  U0=0
  HRBCtrl : Outport
  HRBCtrlBrk : Outport  Port=2
  DecelError : Outport  Port=3
  wires:
  Product/1 -> PI HRB Brake/1(error)
  Product5/1 -> PI HRB Regen/1(error)
  Gain1/1 -> Product5/1  "AccelError"
  Transfer Fcn (with initial outputs)1/1 -> HRBCtrlBrk/1  "HRBCtrlBrk"
  Rset/1 -> Product1/1
  EngineBrkTrqOut/1 -> Add3/1
  wTransOutCmd/1 -> Add/1
  PI HRB Brake/1(ctrl) -> Product2/1  "HRBCtrlBrk"
  wTransOutMeas/1 -> Abs1/1
  Gain2/1 -> Product/1, DecelError/1  "DecelError"
  AccelCmd/1 -> Product5/2
  Saturation1/1 -> Gain2/1
  Saturation2/1 -> Gain1/1
  PI HRB Regen/1(ctrl) -> Add2/2  "HRBCtrlRegen"
  HRBUpEnergyLim/1 -> Product1/2, Product2/2
  Abs1/1 -> Add/2
  DecelCmd/1 -> Product/2
  Product2/1 -> Transfer Fcn (with initial outputs)1/1, Add2/1  "HRBCtrlBrk"
  Add/1 -> Saturation1/1, Saturation2/1  "VehSpdError"
  Transfer Fcn (with initial outputs)/1 -> HRBCtrl/1  "HRBCtrlBrk"
  Constant/1 -> Add3/2
  Product1/1 -> Product/3, PI HRB Brake/2(Rset)  "Rset"
  Add3/1 -> Product5/3
  HRBLoEnergyLim/1 -> Product5/4, PI HRB Regen/2(Rset)
  Add2/1 -> Transfer Fcn (with initial outputs)/1

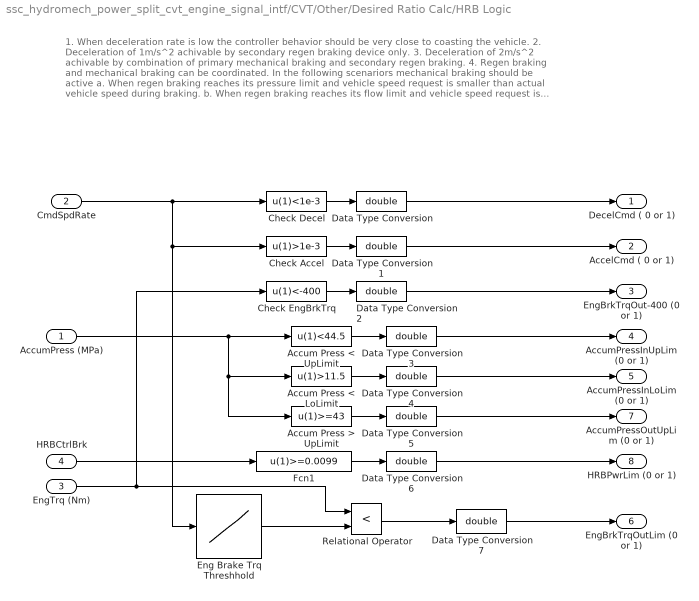
== system ssc_hydromech_power_split_cvt_engine_signal_intf/CVT/Other/Desired Ratio Calc/HRB Logic ==
  note: 1. When deceleration rate is low the controller behavior should be very close to coasting the vehicle.
      | 2. Deceleration of 1m/s^2 achivable by secondary regen braking device only.
      | 3. Deceleration of 2m/s^2 achivable by combination of primary mechanical braking and secondary regen braking.
      | 4. Regen braking and mechanical braking can be coordinated. In the following scenariors mechanical braking should be active
      | a. When regen braking reaches its pressure limit and vehicle speed request is smaller than actual vehicle speed during braking.
      | b. When regen braking reaches its flow limit and vehicle speed request is smaller than actual vehicle speed during braking.
      | 5. Energy in the accumulator will be released when accelerating and the accumulator pressure is above minimum working pressure.
      | Energy release rate should not cause engine over speeding.
      | 6. If engine over speed limit is reached disengage master clutch/shut down the engine.
  AccumPress (MPa) : Inport
  CmdSpdRate : Inport  Port=2
  EngTrq (Nm) : Inport  Port=3
  HRBCtrlBrk : Inport  Port=4
  Accum Press < LoLimit : Fcn  Expr=u(1)>11.5
  Accum Press < UpLimit : Fcn  Expr=u(1)<44.5
  Accum Press > UpLimit : Fcn  Expr=u(1)>=43
  Check Accel : Fcn  Expr=u(1)>1e-3
  Check Decel : Fcn  Expr=u(1)<1e-3
  Check EngBrkTrq : Fcn  Expr=u(1)<-400
  Data Type Conversion{,1..7} (8 alike) : DataTypeConversion  OutDataTypeStr=double  SaturateOnIntegerOverflow=off  RndMeth=Floor
  Eng Brake Trq Threshhold : Lookup_n-D  NumberOfTableDimensions=1  BreakpointsForDimension1=[-3 -2 -1 -0.5 0 1]  Table=[-450 -450 -225 -113 0 0]*0.6  InternalRulePriority=Speed  RndMeth=Simplest
  Fcn1 : Fcn  Expr=u(1)>=0.0099
  Relational Operator : RelationalOperator  Operator=<  OutDataTypeStr=boolean  ZeroCross=off  InputSameDT=off
  DecelCmd ( 0 or 1) : Outport
  AccelCmd ( 0 or 1) : Outport  Port=2
  EngBrkTrqOut-400 (0 or 1) : Outport  Port=3
  AccumPressInUpLim (0 or 1) : Outport  Port=4
  AccumPressInLoLim (0 or 1) : Outport  Port=5
  EngBrkTrqOutLim (0 or 1) : Outport  Port=6
  AccumPressOutUpLim (0 or 1) : Outport  Port=7
  HRBPwrLim (0 or 1) : Outport  Port=8
  wires:
  Check Decel/1 -> Data Type Conversion/1
  Data Type Conversion/1 -> DecelCmd ( 0 or 1)/1
  EngTrq (Nm)/1 -> Relational Operator/1, Check EngBrkTrq/1
  CmdSpdRate/1 -> Check Decel/1, Eng Brake Trq Threshhold/1, Check Accel/1
  Eng Brake Trq Threshhold/1 -> Relational Operator/2
  AccumPress (MPa)/1 -> Accum Press < LoLimit/1, Accum Press > UpLimit/1, Accum Press < UpLimit/1
  Accum Press < UpLimit/1 -> Data Type Conversion3/1
  Relational Operator/1 -> Data Type Conversion7/1
  Accum Press > UpLimit/1 -> Data Type Conversion5/1
  HRBCtrlBrk/1 -> Fcn1/1
  Fcn1/1 -> Data Type Conversion6/1
  Accum Press < LoLimit/1 -> Data Type Conversion4/1
  Check Accel/1 -> Data Type Conversion1/1
  Check EngBrkTrq/1 -> Data Type Conversion2/1
  Data Type Conversion1/1 -> AccelCmd ( 0 or 1)/1
  Data Type Conversion2/1 -> EngBrkTrqOut-400 (0 or 1)/1
  Data Type Conversion3/1 -> AccumPressInUpLim (0 or 1)/1
  Data Type Conversion4/1 -> AccumPressInLoLim (0 or 1)/1
  Data Type Conversion5/1 -> AccumPressOutUpLim (0 or 1)/1
  Data Type Conversion6/1 -> HRBPwrLim (0 or 1)/1
  Data Type Conversion7/1 -> EngBrkTrqOutLim (0 or 1)/1

== system ssc_hydromech_power_split_cvt_engine_signal_intf/CVT/Other/Desired Ratio Calc/MB Control ==
  Decel Error : Inport
  wTransOutCmd : Inport  Port=2
  Rset : Inport  Port=3
  AccumLimUp : Inport  Port=4
  HRBPowerLim : Inport  Port=5
  Add1 : Sum  Inputs=+++
  Compare To Constant : simulink/Logic and Bit Operations/Compare To Constant  relop=<=  const=0.02  OutDataTypeStr=boolean
  Data Type Conversion : DataTypeConversion  OutDataTypeStr=double  SaturateOnIntegerOverflow=off  RndMeth=Floor
  PI MB No HRB : Subsystem
  PI MB with MRB : Subsystem
  Product3 : Product  Inputs=3
  Product4 : Product
  Out1 : Outport
  wires:
  HRBPowerLim/1 -> Product4/2
  AccumLimUp/1 -> Product3/3
  wTransOutCmd/1 -> Compare To Constant/1
  PI MB with MRB/1(ctrl) -> Add1/3
  Add1/1 -> Out1/1
  Product4/1 -> PI MB with MRB/1(error)
  PI MB No HRB/1(ctrl) -> Add1/2
  Data Type Conversion/1 -> Add1/1
  Compare To Constant/1 -> Data Type Conversion/1
  Rset/1 -> PI MB with MRB/2(Rset), PI MB No HRB/2(Rset), Product3/2
  Product3/1 -> PI MB No HRB/1(error)
  Decel Error/1 -> Product4/1, Product3/1

== system ssc_hydromech_power_split_cvt_engine_signal_intf/CVT/Other/Desired Ratio Calc/Subsystem ==
  u : Inport
  Constant1 : Constant
  Constant2 : Constant  Value=-1
  Constant3 : Constant  Value=0
  Gain : Gain  Gain=-1
  Switch : Switch  Criteria=u2 > Threshold  Threshold=0.001  SaturateOnIntegerOverflow=off  InputSameDT=off
  Switch1 : Switch  Criteria=u2 > Threshold  Threshold=0.001  SaturateOnIntegerOverflow=off  InputSameDT=off
  u_dir : Outport
  wires:
  Gain/1 -> Switch1/2
  Switch/1 -> u_dir/1
  u/1 -> Switch/2, Gain/1
  Constant1/1 -> Switch/1
  Switch1/1 -> Switch/3
  Constant3/1 -> Switch1/3
  Constant2/1 -> Switch1/1

== system ssc_hydromech_power_split_cvt_engine_signal_intf/CVT/Other/Port 1 Interface Engine/Interface ==
  across1 : Inport
  across2 : Inport  Port=2
  Continuous : Subsystem  VariantControl=Continuous
  Discrete : Subsystem  VariantControl=Discrete
  through2 : Outport
  through1 : Outport  Port=2

== system ssc_hydromech_power_split_cvt_engine_signal_intf/CVT/Other/Port 1 Interface Vehicle/Interface ==
  across1 : Inport
  across2 : Inport  Port=2
  Continuous : Subsystem  VariantControl=Continuous
  Discrete : Subsystem  VariantControl=Discrete
  through2 : Outport
  through1 : Outport  Port=2

== system ssc_hydromech_power_split_cvt_engine_signal_intf/CVT/Simscape/CVT Ratio Ctrl/Range Calculation ==
  Ratio (-) : Inport
  Check Range 0 or higher : Switch  Threshold=XY_I(1,2)  SaturateOnIntegerOverflow=off  InputSameDT=off
  Check Range 2 or higher : Switch  Threshold=XY_I(2,2)  SaturateOnIntegerOverflow=off  InputSameDT=off
  Check Range 3 or higher : Switch  Threshold=XY_I(3,2)  SaturateOnIntegerOverflow=off  InputSameDT=off
  Check Range 4 : Switch  Threshold=XY_I(4,2)  SaturateOnIntegerOverflow=off  InputSameDT=off
  Constant1 : Constant  Value=2  SampleTime=HMPST.Simu.TimeStep
  Constant2 : Constant  SampleTime=HMPST.Simu.TimeStep
  Constant3 : Constant  Value=-1  SampleTime=HMPST.Simu.TimeStep
  Constant4 : Constant  Value=3  SampleTime=HMPST.Simu.TimeStep
  Constant5 : Constant  Value=4  SampleTime=HMPST.Simu.TimeStep
  Range (-) : Outport
  wires:
  Ratio (-)/1 -> Check Range 0 or higher/2, Check Range 4/2, Check Range 3 or higher/2, Check Range 2 or higher/2
  Constant5/1 -> Check Range 4/1
  Constant4/1 -> Check Range 4/3
  Check Range 4/1 -> Check Range 3 or higher/1
  Constant1/1 -> Check Range 3 or higher/3
  Check Range 3 or higher/1 -> Check Range 2 or higher/1
  Check Range 0 or higher/1 -> Range (-)/1  "Range"
  Constant3/1 -> Check Range 0 or higher/3
  Constant2/1 -> Check Range 2 or higher/3
  Check Range 2 or higher/1 -> Check Range 0 or higher/1

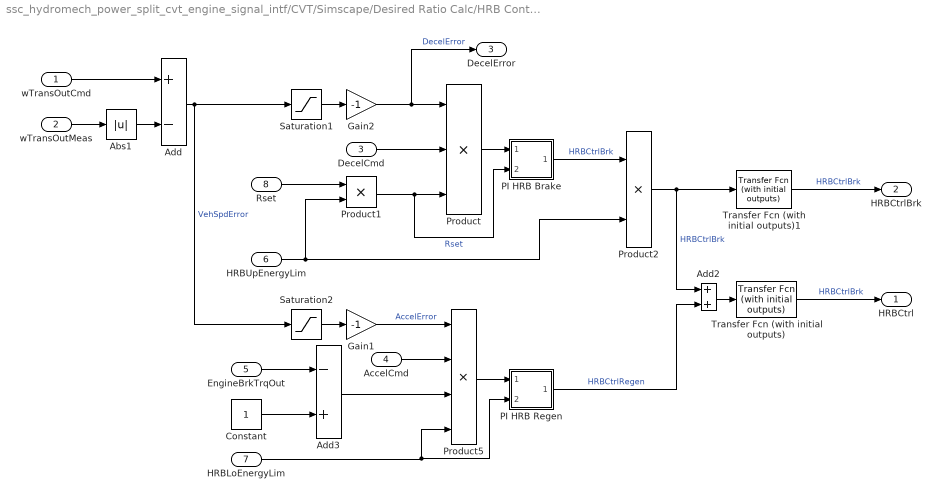
== system ssc_hydromech_power_split_cvt_engine_signal_intf/CVT/Simscape/Desired Ratio Calc/HRB Control ==
  wTransOutCmd : Inport
  wTransOutMeas : Inport  Port=2
  DecelCmd : Inport  Port=3
  AccelCmd : Inport  Port=4
  EngineBrkTrqOut : Inport  Port=5
  HRBUpEnergyLim : Inport  Port=6
  HRBLoEnergyLim : Inport  Port=7
  Rset : Inport  Port=8
  Abs1 : Abs  ZeroCross=off  SaturateOnIntegerOverflow=off
  Add : Sum  Inputs=+-
  Add2 : Sum
  Add3 : Sum  Inputs=-+
  Constant : Constant
  Gain1 : Gain  Gain=-1
  Gain2 : Gain  Gain=-1
  PI HRB Brake : Subsystem
  PI HRB Regen : Subsystem
  Product : Product  Inputs=3
  Product1 : Product
  Product2 : Product
  Product5 : Product  Inputs=4
  Saturation1 : Saturate  UpperLimit=0  LowerLimit=-inf  ZeroCross=off
  Saturation2 : Saturate  UpperLimit=inf  LowerLimit=0  ZeroCross=off
  Transfer Fcn (with initial outputs) : simulink_extras/Additional Linear/Transfer Fcn (with initial outputs)  N=[0.01]  D=[0.05 1]  Y0=0  U0=0
  Transfer Fcn (with initial outputs)1 : simulink_extras/Additional Linear/Transfer Fcn (with initial outputs)  N=[0.01]  D=[0.05 1]  Y0=0  U0=0
  HRBCtrl : Outport
  HRBCtrlBrk : Outport  Port=2
  DecelError : Outport  Port=3
  wires:
  Add2/1 -> Transfer Fcn (with initial outputs)/1
  HRBLoEnergyLim/1 -> PI HRB Regen/2(Rset), Product5/4
  Add3/1 -> Product5/3
  Product1/1 -> PI HRB Brake/2(Rset), Product/3  "Rset"
  Constant/1 -> Add3/2
  Transfer Fcn (with initial outputs)/1 -> HRBCtrl/1  "HRBCtrlBrk"
  Add/1 -> Saturation2/1, Saturation1/1  "VehSpdError"
  Product2/1 -> Add2/1, Transfer Fcn (with initial outputs)1/1  "HRBCtrlBrk"
  DecelCmd/1 -> Product/2
  Abs1/1 -> Add/2
  HRBUpEnergyLim/1 -> Product2/2, Product1/2
  PI HRB Regen/1(ctrl) -> Add2/2  "HRBCtrlRegen"
  Saturation2/1 -> Gain1/1
  Saturation1/1 -> Gain2/1
  AccelCmd/1 -> Product5/2
  Gain2/1 -> DecelError/1, Product/1  "DecelError"
  wTransOutMeas/1 -> Abs1/1
  PI HRB Brake/1(ctrl) -> Product2/1  "HRBCtrlBrk"
  wTransOutCmd/1 -> Add/1
  EngineBrkTrqOut/1 -> Add3/1
  Rset/1 -> Product1/1
  Transfer Fcn (with initial outputs)1/1 -> HRBCtrlBrk/1  "HRBCtrlBrk"
  Gain1/1 -> Product5/1  "AccelError"
  Product5/1 -> PI HRB Regen/1(error)
  Product/1 -> PI HRB Brake/1(error)
